simulink model "simulink_Einspurmodell_COG_linear"  (Simulink 7.6)
settings: Solver=ode5  StartTime=0.0  StopTime=10.0  FixedStep=0.001  RelTol=1e-3
PreLoadFcn:
  | global d
  | global p
undefined symbols (not defined in the file or in its folder): d, int_0, p
settings Model: Creator=tftbe1  LastModifiedBy=TFTBE1
settings DebuggingCC: SaveWithParameterizedLinksMsg=none

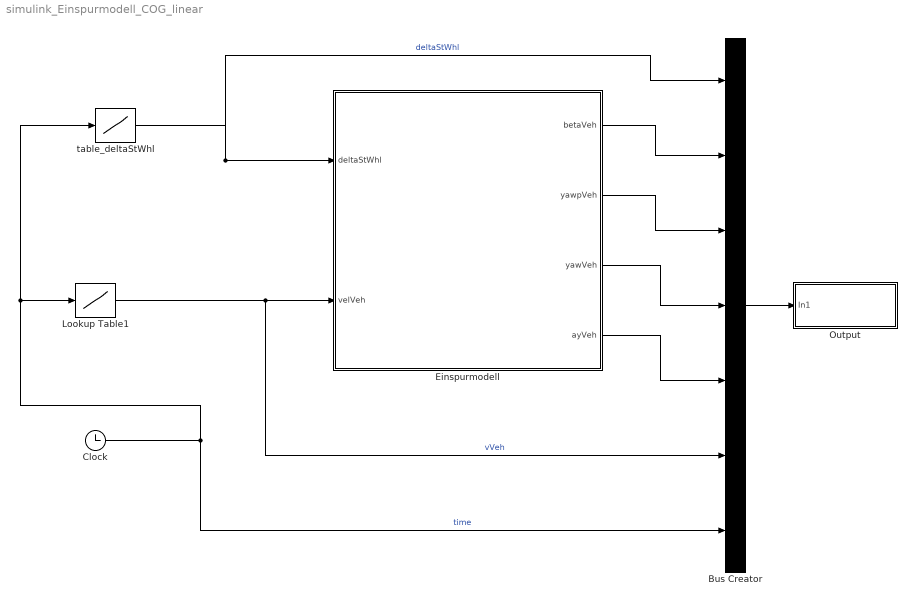
== system simulink_Einspurmodell_COG_linear ==
  Bus Creator : BusCreator  Inputs=7
  Clock : Clock
      settings: Decimation=10
  Einspurmodell : Subsystem
  Lookup Table1 : Lookup  InputValues=d.time  Table=d.vVeh
  Output : Subsystem
  table_deltaStWhl : Lookup  InputValues=d.time  Table=d.deltaStWhl
  wires:
  Bus Creator/1 -> Output/1(In1)
  Einspurmodell/1(betaVeh) -> Bus Creator/2
  Einspurmodell/2(yawpVeh) -> Bus Creator/3
  Einspurmodell/3(yawVeh) -> Bus Creator/4
  Clock/1 -> table_deltaStWhl/1, Lookup Table1/1, Bus Creator/7  "time"
  table_deltaStWhl/1 -> Bus Creator/1, Einspurmodell/1(deltaStWhl)  "deltaStWhl"
  Lookup Table1/1 -> Einspurmodell/2(velVeh), Bus Creator/6  "vVeh"
  Einspurmodell/4(ayVeh) -> Bus Creator/5

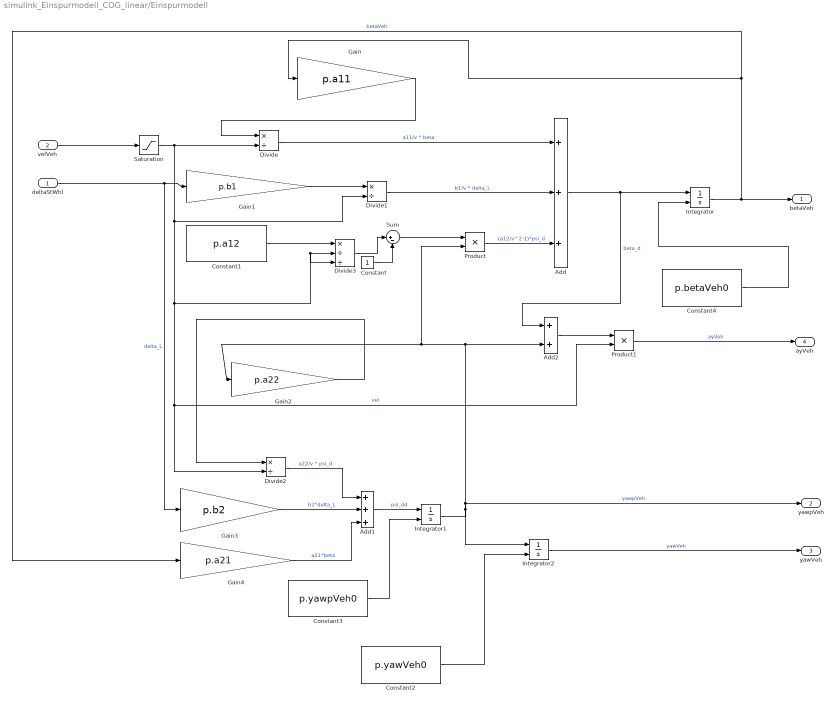
== system simulink_Einspurmodell_COG_linear/Einspurmodell ==
  deltaStWhl : Inport
  velVeh : Inport  Port=2
  Add : Sum  Inputs=+++
  Add1 : Sum  Inputs=+++
  Add2 : Sum
  Constant : Constant
  Constant1 : Constant  Value=p.a12
  Constant2 : Constant  Value=p.yawVeh0
  Constant3 : Constant  Value=p.yawpVeh0
  Constant4 : Constant  Value=p.betaVeh0
  Divide : Product  Inputs=*/
  Divide1 : Product  Inputs=*/
  Divide2 : Product  Inputs=*/
  Divide3 : Product  Inputs=*//
  Gain : Gain  Gain=p.a11
  Gain1 : Gain  Gain=p.b1
  Gain2 : Gain  Gain=p.a22
  Gain3 : Gain  Gain=p.b2
  Gain4 : Gain  Gain=p.a21
  Integrator : Integrator  InitialConditionSource=external  InitialCondition=int_0.beta
  Integrator1 : Integrator  InitialConditionSource=external  InitialCondition=int_0.psi_d
  Integrator2 : Integrator  InitialConditionSource=external  InitialCondition=int_0.psi
  Product : Product  RndMeth=Zero
  Product1 : Product  RndMeth=Zero
  Saturation : Saturate  UpperLimit=inf  LowerLimit=0.1
  Sum : Sum  Inputs=|+-
  betaVeh : Outport
  yawpVeh : Outport  Port=2
  yawVeh : Outport  Port=3
  ayVeh : Outport  Port=4
  wires:
  velVeh/1 -> Saturation/1
  Sum/1 -> Product/1
  Product/1 -> Add/3  "(a12/v^2-1)*psi_d"
  Constant1/1 -> Divide3/1
  Integrator2/1 -> yawVeh/1  "yawVeh"
  Constant/1 -> Sum/2
  Divide3/1 -> Sum/1
  Gain4/1 -> Add1/3  "a21*beta"
  Gain3/1 -> Add1/2  "b2*delta_L"
  Gain2/1 -> Divide2/1
  Divide2/1 -> Add1/1  "a22/v * psi_d"
  Integrator1/1 -> Integrator2/1, yawpVeh/1, Product/2, Gain2/1, Add2/2  "yawpVeh"
  Add1/1 -> Integrator1/1  "psi_dd"
  Gain/1 -> Divide/1
  Divide/1 -> Add/1  "a11/v * beta"
  Divide1/1 -> Add/2  "b1/v * delta_L"
  deltaStWhl/1 -> Gain3/1, Gain1/1  "delta_L"
  Gain1/1 -> Divide1/1
  Saturation/1 -> Divide3/3, Divide3/2, Divide2/2, Product1/2, Divide1/2, Divide/2  "vel"
  Integrator/1 -> betaVeh/1, Gain/1, Gain4/1  "betaVeh"
  Add/1 -> Integrator/1, Add2/1  "beta_d"
  Constant2/1 -> Integrator2/2
  Constant3/1 -> Integrator1/2
  Constant4/1 -> Integrator/2
  Add2/1 -> Product1/1
  Product1/1 -> ayVeh/1  "ayVeh"

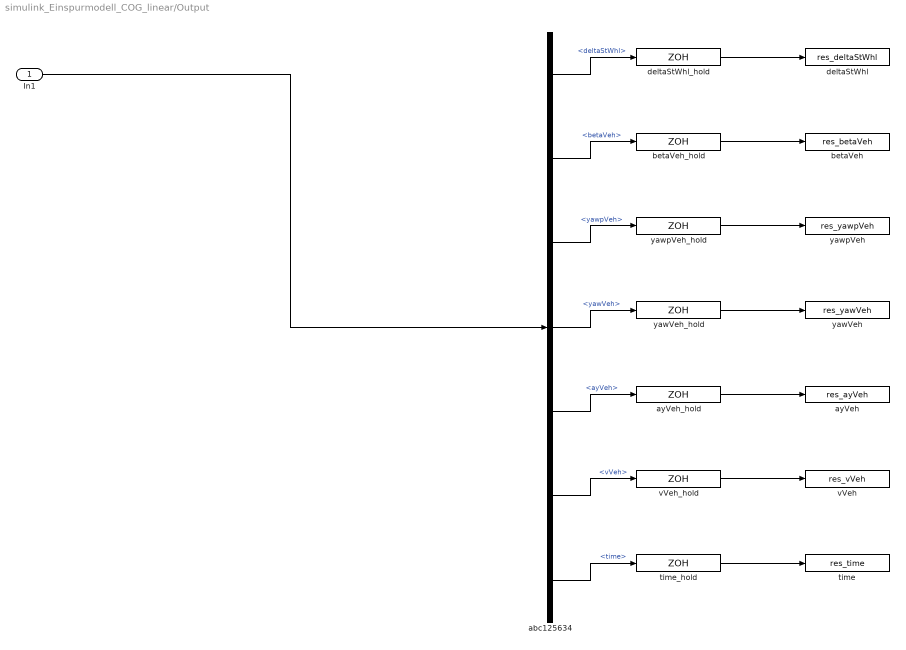
== system simulink_Einspurmodell_COG_linear/Output ==
  In1 : Inport
  abc125634 : BusSelector  OutputSignals=deltaStWhl,betaVeh,yawpVeh,yawVeh,ayVeh,vVeh,time
  ayVeh : ToWorkspace  VariableName=res_ayVeh  SampleTime=-1  SaveFormat=Array
  ayVeh_hold : ZeroOrderHold  SampleTime=0.001
  betaVeh : ToWorkspace  VariableName=res_betaVeh  SampleTime=-1  SaveFormat=Array
  betaVeh_hold : ZeroOrderHold  SampleTime=0.001
  deltaStWhl : ToWorkspace  VariableName=res_deltaStWhl  SampleTime=-1  SaveFormat=Array
  deltaStWhl_hold : ZeroOrderHold  SampleTime=0.001
  time : ToWorkspace  VariableName=res_time  SampleTime=-1  SaveFormat=Array
  time_hold : ZeroOrderHold  SampleTime=0.001
  vVeh : ToWorkspace  VariableName=res_vVeh  SampleTime=-1  SaveFormat=Array
  vVeh_hold : ZeroOrderHold  SampleTime=0.001
  yawVeh : ToWorkspace  VariableName=res_yawVeh  SampleTime=-1  SaveFormat=Array
  yawVeh_hold : ZeroOrderHold  SampleTime=0.001
  yawpVeh : ToWorkspace  VariableName=res_yawpVeh  SampleTime=-1  SaveFormat=Array
  yawpVeh_hold : ZeroOrderHold  SampleTime=0.001
  wires:
  In1/1 -> abc125634/1
  abc125634/1 -> deltaStWhl_hold/1  "<deltaStWhl>"
  deltaStWhl_hold/1 -> deltaStWhl/1
  abc125634/2 -> betaVeh_hold/1  "<betaVeh>"
  betaVeh_hold/1 -> betaVeh/1
  abc125634/3 -> yawpVeh_hold/1  "<yawpVeh>"
  yawpVeh_hold/1 -> yawpVeh/1
  abc125634/4 -> yawVeh_hold/1  "<yawVeh>"
  yawVeh_hold/1 -> yawVeh/1
  abc125634/5 -> ayVeh_hold/1  "<ayVeh>"
  ayVeh_hold/1 -> ayVeh/1
  abc125634/6 -> vVeh_hold/1  "<vVeh>"
  vVeh_hold/1 -> vVeh/1
  abc125634/7 -> time_hold/1  "<time>"
  time_hold/1 -> time/1
